simulink subsystem "Benewake_TF_Luna_8m_LiDAR"  (R2025b)
settings: Solver=VariableStepAuto  StartTime=0.0  StopTime=10.0  RelTol=1e-3
undefined symbols (not defined in the file): dt_lidar, lidar_bias_init, lidar_drift_variance, lidar_max_range, lidar_min_range, lidar_noise_std, lidar_quant_step, lidar_tau
settings Model: Creator=Admin  LastModifiedBy=Admin

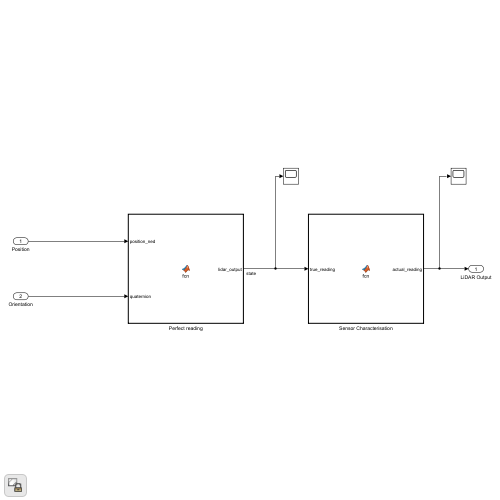
[thumbnail: Simulink's stored preview of the top-level diagram]
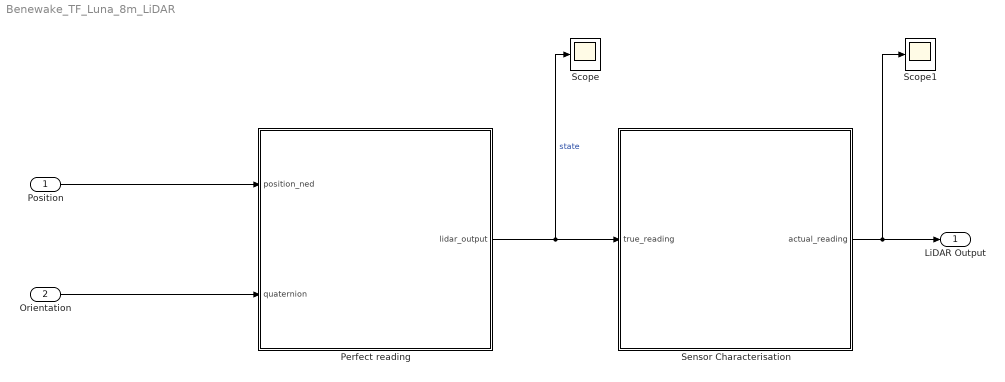
== system Benewake_TF_Luna_8m_LiDAR ==
  Position : Inport
  Orientation : Inport  Port=2
  Perfect reading : MATLAB Function  TreatAsAtomicUnit=on
  Scope : Scope
      settings: ActiveDisplayYMinimum=-0.24999999999999994  ActiveDisplayYMaximum=2.25
  Scope1 : Scope
      settings: ActiveDisplayYMinimum=-1  ActiveDisplayYMaximum=1
  Sensor Characterisation : MATLAB Function  TreatAsAtomicUnit=on
  LiDAR Output : Outport
  wires:
  Sensor Characterisation/1(actual_reading) -> LiDAR Output/1, Scope1/1
  Perfect reading/1(lidar_output) -> Sensor Characterisation/1(true_reading), Scope/1  "state"
  Orientation/1 -> Perfect reading/2(quaternion)
  Position/1 -> Perfect reading/1(position_ned)

== matlab function Benewake_TF_Luna_8m_LiDAR/Sensor Characterisation ==
  settings: updateMethod=DISCRETE  sampleTime=dt_lidar
  data: true_reading input; actual_reading output; dt_lidar parameter double size=1; lidar_bias_init parameter double size=1; lidar_tau parameter double size=1; lidar_drift_variance parameter double size=1; lidar_noise_std parameter double size=1; lidar_quant_step parameter double size=1; lidar_min_range parameter double size=1; lidar_max_range parameter double size=1
function actual_reading=fcn(true_reading,dt_lidar,lidar_bias_init,lidar_tau,lidar_drift_variance,lidar_noise_std,lidar_quant_step,lidar_min_range,lidar_max_range)
%#codegen
% actual_reading=[range_m;valid_flag]
% Ignore range_m when valid_flag=0.

persistent b_previous

if isempty(b_previous)
    b_previous=0;
end

tau=max(lidar_tau,1e-9);
q=max(lidar_drift_variance,0);

% First-order Gauss-Markov drift
phi=exp(-dt_lidar/tau);
omega=sqrt(q)*randn;
b_drift=phi*b_previous+omega;
b_previous=b_drift;

% Bias and white noise
composite_bias=lidar_bias_init+b_drift;
noise=lidar_noise_std*randn;

% Default: invalid measurement with a finite placeholder
actual_reading=[0;0];

% Reject missing returns and true ranges outside sensor limits
if ~isfinite(true_reading) || ...
        true_reading<lidar_min_range || ...
        true_reading>lidar_max_range
    return;
end

% Add measurement errors and quantize without clamping
unquantised_reading=true_reading+composite_bias+noise;
quantised_reading=lidar_quant_step* ...
    round(unquantised_reading/lidar_quant_step);

% Accept only finite measured ranges within sensor limits
if isfinite(quantised_reading) && ...
        quantised_reading>=lidar_min_range && ...
        quantised_reading<=lidar_max_range
    actual_reading=[quantised_reading;1];
end

end

== matlab function Benewake_TF_Luna_8m_LiDAR/Perfect reading ==
  data: position_ned input; lidar_output output; quaternion input
function lidar_output = fcn(position_ned, quaternion)
%#codegen
% position_ned: [North;East;Down], metres
% quaternion: scalar-first, NED-to-body convention
% Assumptions:
% - ground is the NED plane Down = 0
% - LiDAR points along body -X

position_ned = position_ned(:);
quaternion = quaternion(:);

q_norm = norm(quaternion);

if q_norm < 1e-12
    lidar_output = Inf;
    return;
end

quaternion = quaternion ./ q_norm;

% Downward-facing LiDAR direction in body axes
beam_body = [-1;0;0];

% Express beam direction in NED
beam_ned = body2ned(beam_body, quaternion);
beam_ned = beam_ned ./ norm(beam_ned);

beam_down = beam_ned(3);
position_down = position_ned(3);

% Beam is horizontal or pointing upward
if beam_down <= 1e-6
    lidar_output = Inf;
    return;
end

% Intersection with ground plane Down = 0
lidar_output = -position_down / beam_down;

% Ground is behind the sensor
if lidar_output < 0
    lidar_output = Inf;
end

end
